simulink model "flightControlSystem"  (R2026a)
settings: Solver=ode3  StartTime=0  FixedStep=Ts  EnableMultiTasking=on
settings Model: Creator=The MathWorks, Inc.  LastModifiedBy=The MathWorks, Inc.
settings OptimizationCC: BufferReuse=off
settings DebuggingCC: SymbolicDimsDataTypeCodeGenerationDiagnostic=none
settings HardwareCC: ProdHWDeviceType=32-bit Generic

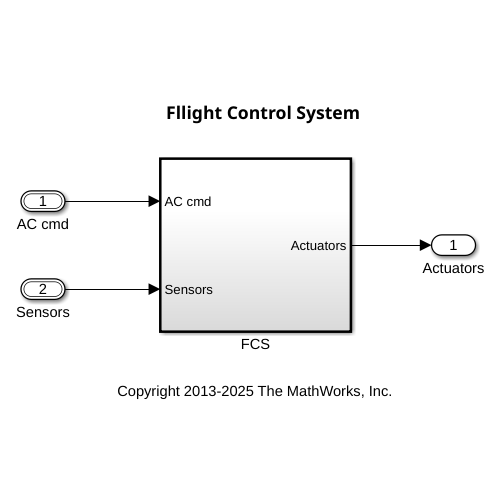
[thumbnail: Simulink's stored preview of the top-level diagram]
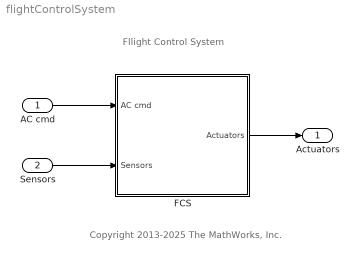
== system flightControlSystem ==
  note: Copyright 2013-2025 The MathWorks, Inc.
  note: Fllight Control System
  AC cmd : Inport  OutDataTypeStr=Bus: CommandBus  BusOutputAsStruct=on
  Sensors : Inport  Port=2  OutDataTypeStr=Bus: SensorsBus  BusOutputAsStruct=on
  FCS : Subsystem  TreatAsAtomicUnit=on
  Actuators : Outport  VectorParamsAs1DForOutWhenUnconnected=off
  wires:
  AC cmd/1 -> FCS/1(AC cmd)
  Sensors/1 -> FCS/2(Sensors)
  FCS/1(Actuators) -> Actuators/1

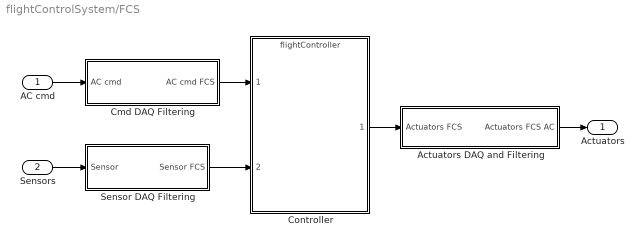
== system flightControlSystem/FCS ==
  AC cmd : Inport
  Sensors : Inport  Port=2
  Actuators DAQ and Filtering : Subsystem
  Cmd DAQ Filtering : Subsystem
  Controller : ModelReference  ModelNameDialog=flightController.slx  SimulationMode=Normal  ModelReferenceVersion=13.0
  Sensor DAQ Filtering : Subsystem
  Actuators : Outport  VectorParamsAs1DForOutWhenUnconnected=off
  wires:
  Sensor DAQ Filtering/1(Sensor FCS) -> Controller/2
  Controller/1 -> Actuators DAQ and Filtering/1(Actuators FCS)
  AC cmd/1 -> Cmd DAQ Filtering/1(AC cmd)
  Actuators DAQ and Filtering/1(Actuators FCS AC) -> Actuators/1
  Sensors/1 -> Sensor DAQ Filtering/1(Sensor)
  Cmd DAQ Filtering/1(AC cmd FCS) -> Controller/1

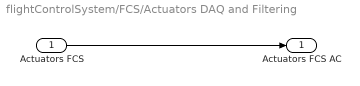
== system flightControlSystem/FCS/Actuators DAQ and Filtering ==
  Actuators FCS : Inport
  Actuators FCS AC : Outport  VectorParamsAs1DForOutWhenUnconnected=off
  wires:
  Actuators FCS/1 -> Actuators FCS AC/1

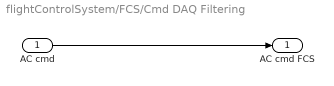
== system flightControlSystem/FCS/Cmd DAQ Filtering ==
  AC cmd : Inport
  AC cmd FCS : Outport  VectorParamsAs1DForOutWhenUnconnected=off
  wires:
  AC cmd/1 -> AC cmd FCS/1

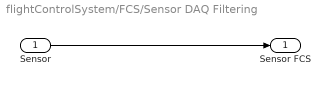
== system flightControlSystem/FCS/Sensor DAQ Filtering ==
  Sensor : Inport
  Sensor FCS : Outport  VectorParamsAs1DForOutWhenUnconnected=off
  wires:
  Sensor/1 -> Sensor FCS/1
